simulink model "turbo_controller"  (R2025a)
settings: Solver=FixedStepAuto  StartTime=0.0  StopTime=inf  FixedStep=0.001  RelTol=1e-3
PostLoadFcn:
  | % 自动定位同目录CubeMX文件；不需要外部初始化脚本。
  | codertarget.data.setParameterValue('turbo_controller','STM32CubeMX.ProjectFile',fullfile(fileparts(get_param('turbo_controller','FileName')),'turbo_f407.ioc'));
InitFcn:
  | % 中文说明：按原控制器字段与类型创建三组接口总线；控制参数已内嵌。
  | tc_names=["EValve_Cycle" "EValve_Open" "Eblast_Cycle" "Eblast_Open" "Motor_Cycle" "Motor_Open" "EValve_Enable" "Eblast_Enable" "Motor_Enable" "SWO_Firework" "SWO_BleedAir" "EngineState" "Flag_ECUReset_Clear" "Flag_ECUReset_Save" "Flag_Reset_Enable" "Accelerator" "Nc_dem" "Nc"]; tc_types=["uint16" "uint16" "uint16" "uint16" "uint16" "uint16" "uint8" "uint8" "uint8" "uint8" "uint8" "uint8" "uint8" "uint8" "uint8" "single" "single" "single"];
  | for tc_k=1:numel(tc_names)
  |  tc_e(tc_k)=Simulink.BusElement; tc_e(tc_k).Name=char(tc_names(tc_k)); tc_e(tc_k).DataType=char(tc_types(tc_k));
  | end
  | EngineControl_Out=Simulink.Bus; EngineControl_Out.DataScope='Exported'; EngineControl_Out.Elements=tc_e;
  | clear tc_e tc_names tc_types tc_k
  | tc_names=["savedata1" "savedata2" "savedata3" "savedata4" "savedata5" "savedata6" "savedata7" "savedata8" "savedata9" "savedata10" "savedata11" "savedata12" "savedata13" "savedata14" "savedata15" "savedata16" "savedata17" "savedata18" "savedata19" "savedata20" "savedata21" "savedata22" "savedata23" "savedata24" "savedata25"]; tc_types=["single" "single" "single" "single" "single" "single" "single" "single" "single" "single" "single" "single" "single" "single" "single" "single" "single" "single" "single" "single" "single" "single" "single" "single" "single"];
  | for tc_k=1:numel(tc_names)
  |  tc_e(tc_k)=Simulink.BusElement; tc_e(tc_k).Name=char(tc_names(tc_k)); tc_e(tc_k).DataType=char(tc_types(tc_k));
  | end
  | SaveData_Out=Simulink.Bus; SaveData_Out.DataScope='Exported'; SaveData_Out.Elements=tc_e;
  | clear tc_e tc_names tc_types tc_k
  | tc_names=["senddata1" "senddata2" "senddata3" "senddata4" "senddata5" "senddata6" "senddata7" "senddata8" "senddata9" "senddata10" "senddata11" "senddata12" "senddata13" "senddata14" "senddata15" "senddata16" "senddata17" "senddata18" "senddata19" "senddata20" "senddata21" "senddata22" "senddata23" "senddata24" "senddata25" "senddata26" "senddata27" "senddata28" "senddata29"]; tc_types=["uint8" "uint8" "uint8" "uint8" "uint8" "uint8" "uint8" "uint8" "uint8" "uint8" "uint8" "uint8" "uint8" "uint8" "uint8" "uint8" "uint8" "uint8" "uint8" "uint8" "uint8" "uint8" "uint8" "uint8" "uint8" "uint8" "uint8" "uint8" "uint8"];
  | for tc_k=1:numel(tc_names)
  |  tc_e(tc_k)=Simulink.BusElement; tc_e(tc_k).Name=char(tc_names(tc_k)); tc_e(tc_k).DataType=char(tc_types(tc_k));
  | end
  | SendData_Out=Simulink.Bus; SendData_Out.DataScope='Exported'; SendData_Out.Elements=tc_e;
  | clear tc_e tc_names tc_types tc_k
  | 
  | % 以下为接口中文说明；只设置描述，不改变数值或数据类型。
  | EngineControl_Out.Description='执行控制输出（阀、电机、点火、状态及复位请求）';
  | tc_cn=["EValve_Cycle（主油阀周期计数（每计数2毫秒））" "EValve_Open（主油阀开通计数（每计数2毫秒））" "Eblast_Cycle（副油阀周期计数（每计数2毫秒））" "Eblast_Open（副油阀开通计数（每计数2毫秒））" "Motor_Cycle（起动电机周期计数）" "Motor_Open（起动电机开通计数）" "EValve_Enable（主油阀驱动使能）" "Eblast_Enable（副油阀驱动使能）" "Motor_Enable（起动电机使能）" "SWO_Firework（点火器使能（1开））" "SWO_BleedAir（引气阀使能（1开））" "EngineState（发动机状态）" "Flag_ECUReset_Clear（清除复位恢复状态请求）" "Flag_ECUReset_Save（保存复位恢复数据请求）" "Flag_Reset_Enable（处理器软件复位请求）" "Accelerator（油门／油泵给定控制量）" "Nc_dem（控制目标转速）" "Nc（发动机反馈转速（转每分））"];
  | tc_elements=EngineControl_Out.Elements;
  | for tc_k=1:numel(tc_cn)
  |  tc_elements(tc_k).Description=char(tc_cn(tc_k));
  | end
  | EngineControl_Out.Elements=tc_elements;
  | clear tc_cn tc_elements tc_k
  | SaveData_Out.Description='25项运行记录；字段含义按当前模型数据来源解释';
  | tc_cn=["savedata1（指令回显记录）" "savedata2（入口总温记录（℃））" "savedata3（电源电压记录）" "savedata4（排气温度记录（℃））" "savedata5（标定燃油压力记录）" "savedata6（副油阀占空比记录（％））" "savedata7（主油阀占空比记录（％））" "savedata8（温度修正转速记录）" "savedata9（开关输出及反馈位域）" "savedata10（物理转速记录）" "savedata11（油泵目标给定原始值）" "savedata12（起动电机占空比记录（％））" "savedata13（发动机状态码记录）" "savedata14（故障告警位域记录）" "savedata15（模型记录帧序号）" "savedata16（处理器温度记录（℃））" "savedata17（装订转速记录（沿用旧电源字段名））" "savedata18（导航高度记录）" "savedata19（飞行空速记录）" "savedata20（主阀旧记录位（恒零保留））" "savedata21（第21项保留记录（恒零））" "savedata22（保留记录项22）" "savedata23（保留记录项23）" "savedata24（保留记录项24）" "savedata25（保留记录项25）"];
  | tc_elements=SaveData_Out.Elements;
  | for tc_k=1:numel(tc_cn)
  |  tc_elements(tc_k).Description=char(tc_cn(tc_k));
  | end
  | SaveData_Out.Elements=tc_elements;
  | clear tc_cn tc_elements tc_k
  | SendData_Out.Description='29字段回传及外设命令接口；板端上位机帧只取第3至27字段';
  | tc_cn=["senddata1（回传发送允许标志（不直接上线路））" "senddata2（回传载荷长度25字节）" "senddata3（回传指令回显字节）" "senddata4（总温编码字节（℃＋80））" "senddata5（电源电压编码字节）" "senddata6（排温编码高字节）" "senddata7（排温编码低字节）" "senddata8（燃油压力编码高字节）" "senddata9（燃油压力编码低字节）" "senddata10（副油阀占空比字节（％））" "senddata11（主油阀占空比字节（％））" "senddata12（修正转速编码高字节）" "senddata13（修正转速编码低字节）" "senddata14（驱动及反馈状态位域）" "senddata15（物理转速编码高字节）" "senddata16（物理转速编码低字节）" "senddata17（油泵目标给定高字节（串口二使用））" "senddata18（油泵目标给定低字节（串口二使用））" "senddata19（起动电机占空比命令（串口一使用））" "senddata20（发动机状态码字节）" "senddata21（故障告警位域字节）" "senddata22（帧序号占位（板端另行填写））" "senddata23（处理器温度编码（℃＋50））" "senddata24（控制目标转速编码高字节）" "senddata25（控制目标转速编码低字节）" "senddata26（占位字节（板端改填实测泵速高字节））" "senddata27（占位字节（板端改填实测泵速低字节））" "senddata28（装订转速高字节（本板未发送））" "senddata29（装订转速低字节（本板未发送））"];
  | tc_elements=SendData_Out.Elements;
  | for tc_k=1:numel(tc_cn)
  |  tc_elements(tc_k).Description=char(tc_cn(tc_k));
  | end
  | SendData_Out.Elements=tc_elements;
  | clear tc_cn tc_elements tc_k
  | 
  | 
  | % FRAM模块化事务：接口类型和上电初始状态，随模型保存，无外部初始化文件。
  | clear FM_elements
  | FM_elements(1)=Simulink.BusElement;FM_elements(1).Name='phase';FM_elements(1).DataType='uint8';FM_elements(1).Dimensions=[1 1];FM_elements(1).Description='phase（当前事务阶段）';
  | FM_elements(2)=Simulink.BusElement;FM_elements(2).Name='a';FM_elements(2).DataType='uint8';FM_elements(2).Dimensions=[64 1];FM_elements(2).Description='a（启动时缓存的首区64字节）';
  | FM_elements(3)=Simulink.BusElement;FM_elements(3).Name='active';FM_elements(3).DataType='uint16';FM_elements(3).Dimensions=[1 1];FM_elements(3).Description='active（当前有效记录区地址）';
  | FM_elements(4)=Simulink.BusElement;FM_elements(4).Name='generation';FM_elements(4).DataType='uint32';FM_elements(4).Dimensions=[1 1];FM_elements(4).Description='generation（当前有效记录代号）';
  | FM_elements(5)=Simulink.BusElement;FM_elements(5).Name='record';FM_elements(5).DataType='uint8';FM_elements(5).Dimensions=[64 1];FM_elements(5).Description='record（本次冻结的待写记录）';
  | FM_elements(6)=Simulink.BusElement;FM_elements(6).Name='addr';FM_elements(6).DataType='uint16';FM_elements(6).Dimensions=[1 1];FM_elements(6).Description='addr（本次备用写入地址）';
  | FM_elements(7)=Simulink.BusElement;FM_elements(7).Name='lastSave';FM_elements(7).DataType='single';FM_elements(7).Dimensions=[1 1];FM_elements(7).Description='lastSave（上次开始保存的秒数）';
  | FM_elements(8)=Simulink.BusElement;FM_elements(8).Name='lastState';FM_elements(8).DataType='uint8';FM_elements(8).Dimensions=[1 1];FM_elements(8).Description='lastState（上次保存时的发动机状态）';
  | FM_elements(9)=Simulink.BusElement;FM_elements(9).Name='boot';FM_elements(9).DataType='boolean';FM_elements(9).Dimensions=[1 1];FM_elements(9).Description='boot（启动记录是否允许恢复）';
  | FM_elements(10)=Simulink.BusElement;FM_elements(10).Name='consumed';FM_elements(10).DataType='boolean';FM_elements(10).Dimensions=[1 1];FM_elements(10).Description='consumed（本次启动恢复通知是否已发送）';
  | FM_elements(11)=Simulink.BusElement;FM_elements(11).Name='payload';FM_elements(11).DataType='uint8';FM_elements(11).Dimensions=[20 1];FM_elements(11).Description='payload（当前20字节恢复内容）';
  | ... (+35 lines)
model workspace (MAT data in the model file):
  CRC16_Table_Reference = [0 4129 8258 12387 16516 20645 24774 28903 33032 37161 41290 45419 ... (256 elements, 256x1)]
  PE_Kaer = [0.15402 0.15402 0.12264 0.10076 0.09481 0.07601 0.07111 0.0569 0.05198 0.04926 0.05308 0.04325 ... (13 elements, 1x13)]
  PE_Nr = [21.2982 61.4260372 67.7475458 72.7394382 76.845934 80.6988798 83.8449282 86.6491912 88.9382406 89.178606 91.1938214 93.4068058 ... (13 elements, 1x13)]
  PE_Pump_Translate = 33.5999984741
  PE_RotaSpeed_Translate = 860
  PE_Taer = [0.4939154 0.4939154 0.40780982 0.34066978 0.31622756 0.30405716 0.34300244 0.26785022 0.37393554 0.23914836 0.44563948 0.31044662 ... (13 elements, 1x13)]
  PF_ACCFULLRANGE = 3360
  PF_Flag_ECUReset = 0
  PF_Flag_rx_suc = 1
  PF_Gear_Info = [40000; 45000; 50000; 55000; 57000; 59000; 60000; 61000; 61000; 61000; 61000; 61000]
  PF_K_TiaoJie = 1
  PF_Kpu = 10
  PF_MySet_Rxdata = [0 0 0 0 0 0 0 0 0 0 0 0 ... (50 elements, 50x1)]
  PF_MyUsart1_Rxdata = [0 0 0 0 0 0 0 0 0 0 0 0 ... (50 elements, 50x1)]
  PF_MyUsart2_Rxdata = [0 0 0 0 0 0 0 0 0 0 0 0 ... (50 elements, 50x1)]
  PF_Reset_Information = [0 0 0 0 0 0 0 0 0 0 0 0 ... (20 elements, 20x1)]
  PF_Sensor_X1_T4 = [0 4095]
  PF_Sensor_X2_T4 = [0 1.66666698456]
  PF_Sensor_X3_T4 = [0 504 999 1497 2010 2529 3051 3568 4076 4571 4959]
  PF_Sensor_X_P2 = [0.5 3]
  PF_Sensor_X_Poil = [0.5 3]
  PF_Sensor_X_T1t = [-50 300]
  PF_Sensor_X_Vpower = [0 3]
  PF_Sensor_X_Vpump = [0 3]
  PF_Sensor_Y1_T4 = [0 3]
  PF_Sensor_Y2_T4 = [0 5000]
  PF_Sensor_Y3_T4 = [0 100 200 300 400 500 600 700 800 900 980]
  PF_Sensor_Y_P2 = [0 1000]
  PF_Sensor_Y_Poil = [0 1000]
  PF_Sensor_Y_T1t = [-50 300]
  PF_Sensor_Y_Vpower = [0 33]
  PF_Sensor_Y_Vpump = [0 33]
  PG_CtrlMode_CloseLoop : mpt.Parameter (value not decoded)
  PG_CtrlMode_ManualAcc : mpt.Parameter (value not decoded)
  PG_CtrlMode_Origin : mpt.Parameter (value not decoded)
  PG_CtrlMode_Start : mpt.Parameter (value not decoded)
  PG_CtrlMode_Stop : mpt.Parameter (value not decoded)
  PG_ES_Clp : mpt.Parameter (value not decoded)
  PG_ES_EngStart : mpt.Parameter (value not decoded)
  PG_ES_Manual : mpt.Parameter (value not decoded)
  PG_ES_Origin : mpt.Parameter (value not decoded)
  PG_ES_Stop : mpt.Parameter (value not decoded)
  PG_Instr_BleedAirSet : mpt.Parameter (value not decoded)
  PG_Instr_CloseLoop : mpt.Parameter (value not decoded)
  PG_Instr_ECUReSet : mpt.Parameter (value not decoded)
  PG_Instr_EValveSet : mpt.Parameter (value not decoded)
  PG_Instr_EblastSet : mpt.Parameter (value not decoded)
  PG_Instr_Erase : mpt.Parameter (value not decoded)
  PG_Instr_FireWorkSet : mpt.Parameter (value not decoded)
  PG_Instr_ManualPlus : mpt.Parameter (value not decoded)
  PG_Instr_ManualrReduce : mpt.Parameter (value not decoded)
  PG_Instr_MotorSet : mpt.Parameter (value not decoded)
  PG_Instr_OilSet : mpt.Parameter (value not decoded)
  PG_Instr_SelfCheck : mpt.Parameter (value not decoded)
  PG_Instr_Start : mpt.Parameter (value not decoded)
  PG_Instr_Stop : mpt.Parameter (value not decoded)
  PG_Instr_StopZero : Simulink.Parameter (value not decoded)
  PG_Location_Air : Simulink.Parameter (value not decoded)
  PG_Location_Gnd : Simulink.Parameter (value not decoded)
  PG_ServoCtrlMode_CloseLoop : Simulink.Parameter (value not decoded)
  PG_ServoCtrlMode_CloseLoopMax : Simulink.Parameter (value not decoded)
  PG_ServoCtrlMode_CloseLoopMin : Simulink.Parameter (value not decoded)
  PG_ServoCtrlMode_ManualAcc : Simulink.Parameter (value not decoded)
  PG_ServoCtrlMode_ManualAccMax : Simulink.Parameter (value not decoded)
  PG_ServoCtrlMode_ManualAccMin : Simulink.Parameter (value not decoded)
  PG_SpeedDot_Permit : Simulink.Parameter (value not decoded)
  PL_EngineModel_Actuator = [0 10 100]
  PL_EngineModel_EngineStar_Press_P2 = [1013 1098.4 1099.144828 1099.931034 1103.613793 1162.662069 1143.793103 1131.006897 1123.186207 1117.6 1114 1111.806897 ... (127 elements, 1x127)]
  PL_EngineModel_EngineStar_RotaSpeed = [200 2000 9584 9660 10220 10240 10260 10288 10308 10368 10380 10408 ... (127 elements, 1x127)]
  PL_EngineModel_EngineStar_Temp_Exhaust = [128 129 129.1 130 131 131.1 132 133 134 134.1 135 135.1 ... (127 elements, 1x127)]
  PL_EngineModel_EngineStar_Time = [0.05 0.1 0.15 0.2 0.25 0.3 0.35 0.4 0.45 0.5 0.55 0.6 ... (127 elements, 1x127)]
  PL_EngineModel_IdleAbove_Nr = [0 21.2982 61.4260372 67.7475458 72.7394382 76.845934 80.6988798 83.8449282 86.6491912 88.9382406 89.178606 91.1938214 ... (14 elements, 1x14)]
  PL_EngineModel_IdleAbove_P2r = [0.986923266716 1.57907722675 1.81593881076 1.99358499877 2.23044658278 2.43770046879 2.65482358747 2.84233900814 3.03972366149 3.18776215149 3.25684678016 3.3950160375 ... (14 elements, 1x14)]
  PL_EngineModel_IdleAbove_Tempr = [0.0536001429337 1.07200285867 1.63301768805 1.63659103091 1.66875111667 1.72592460247 1.77595140254 1.86171163123 1.95461854565 2.03323208862 2.03323208862 2.13685903162 ... (14 elements, 1x14)]
  PL_EngineModel_IdleAbove_Ter = [0.42434128 0.42434128 0.42434128 0.30669408 0.23570008 0.22150128 0.1997974 0.23803274 0.16115638 0.24279948 0.13600422 0.31308354 ... (14 elements, 1x14)]
  PL_EngineModel_IdleAbove_Wfr = [0 10.142 23.8337 27.8905 31.9473 36.0041 40.0609 44.1177 48.1745 52.2313 52.7384 56.7952 ... (14 elements, 1x14)]
  PL_EngineModel_Press_P2 = [400 400 400 400 400 400 400 400 400 400]
  PL_EngineModel_Rotaspeed = [0 20000 96400]
  PL_EngineModel_Temp_Exhaust = [500 500 500 500 500 500 500 500 500 500]
  PL_Kaer = [0.1 0.1 0.1 0.1 0.1 0.1]
  PL_Nr = [50 60 70 80 90 100]
  PL_Taer = [0.1 0.1 0.1 0.1 0.1 0.1]
  Sig : Simulink.Signal (value not decoded)
  Ts_ms : Simulink.Parameter (value not decoded)
  false : Simulink.Parameter (value not decoded)
  true : Simulink.Parameter (value not decoded)
symbols that are objects in the model workspace (value not decoded): PG_CtrlMode_CloseLoop, PG_CtrlMode_ManualAcc, PG_CtrlMode_Origin, PG_CtrlMode_Start, PG_CtrlMode_Stop, PG_ES_Clp, PG_ES_EngStart, PG_ES_Manual, PG_ES_Origin, PG_ES_Stop, PG_Instr_BleedAirSet, PG_Instr_CloseLoop, PG_Instr_EblastSet, PG_Instr_ECUReSet, PG_Instr_Erase, PG_Instr_EValveSet, PG_Instr_FireWorkSet, PG_Instr_ManualPlus, PG_Instr_ManualrReduce, PG_Instr_MotorSet, PG_Instr_OilSet, PG_Instr_SelfCheck, PG_Instr_Start, PG_Instr_Stop, PG_Instr_StopZero, PG_ServoCtrlMode_CloseLoop, PG_ServoCtrlMode_CloseLoopMax, PG_ServoCtrlMode_CloseLoopMin, PG_ServoCtrlMode_ManualAcc, PG_ServoCtrlMode_ManualAccMax, PG_ServoCtrlMode_ManualAccMin, Ts_ms
libraries: simulink x97, stm32blockslib x10, stm32f4xxblockslib x8
(part 19 of 26)

== system turbo_controller/BoardOutput_串口封装与阀门时序/Out04_Command（电机及油泵指令）/PumpFrame（油泵指令使用原高低给定字节）_973/CRC16（只校验两个命令字节）_961 ==
  note: 【中文学习说明：CRC16查表法】
      | 一、大白话：把逐位算出的答案预先放进表里。
      | 收到每个字节后，用旧校验值和当前字节算一个表下标，
      | 直接查出结果，再与旧值左移一个字节后的部分异或。
      | 每字节只查一次表，不再进行8次逐位循环。
      |
      | 二、本模块一次处理2个数据字节。
      | 每帧校验值从0开始；逐字节循环仍按输入顺序执行。
      | 先将当前字节放到高八位，与旧CRC异或，
      | 再交给TableStep（查表更新）算出新CRC，
      | 记住新CRC后处理下一个字节，最后输出16位结果。
      |
      | 三、和参考工程逐项对应。
      | 参考写法：index=((旧CRC>>8) XOR 当前字节) AND 255。
      | 新CRC=表[index] XOR ((旧CRC<<8) AND 65535)。
      | 本图先合并字节再取高八位，得到完全相同的index。
      | 表为参考工程crc.c中的原始256项uint16数据，
      | 保存在模型工作区CRC16_Table_Reference中，
      | 所有CRC16模块使用同一份表，无需额外源文件。
      |
      | 四、协议规则没有改变。
      | 初值0、多项式0x1021、高位先处理、不作末尾异或。
      | 校验范围由外层选取，帧头和帧尾校验字节不随意加入。
      | 输出仍由外层拆成高、低字节，高字节在前。
      | 这里只计算CRC，是否采纳数据由外层校验比较决定。
      |
      | 五、记忆与循环要分清。
      | 外层逐字节循环在一次调用内处理整段数据，
      | 并非每处理一字节就等待一个采样周期。
      | CRC记忆块传递同一帧中上一个字节的结果；
      | 每次重新计算一帧时从0开始，不串用上一帧的结果。
      | 查表能发现传输错误，不能修复数据，也不是加密。
  note: 整段字节如何逐个累积CRC16
      |
      | 这里的输入Bytes是发给外设的两个命令字节，不含前五项帧头。CRC的作用是把整段字节压缩成一个16
      | 位检查值，便于接收方发现传输内容变化。
      |
      | 每帧从初始CRC=uint16(0)开始。循环一次取一个字节，把该字节乘256移到高8位，与旧CRC异或，得到
      | Merged，再交给TableStep执行查表移位。TableStep的输出成为处理下一个字节的旧CRC。
      |
      | 公式第一步是Merged=bitxor(旧CRC,当前字节×256)。整个循环结束后输出最后一次CRC，父级拆成高、
      | 低字节用于比较或发送。For Iterator中的CRC记忆是帧内累积状态，不能理解成跨帧无限累加。
      |
      | 这里用的是CRC16_Table_Reference指定的算法表，不能随意换另一种CRC表或初始值。相同字节、顺序
      | 、表和初值必须得到相同结果，双方才能校验通过。
  Bytes（待校验字节）_931 : Inport  OutDataTypeStr=uint8
  CRC（本帧累计校验值）_933 : UnitDelay  InitialCondition=uint16(0)  SampleTime=-1  HasFrameUpgradeWarning=on
  Cast（数据类型转换）_935 : DataTypeConversion  OutDataTypeStr=uint16  RndMeth=Round
  Constant（常量）_936 : Constant  Value=256  OutDataTypeStr=uint16
  CurrentByte（当前字节）_934 : Selector  InputPortWidth=2  IndexOptions=Index vector (port)  Indices=1  OutputSizes=1
  EachByte（逐字节校验）_932 : ForIterator  ResetStates=reset  IterationLimit=2  IterationVariableDataType=uint32
  HighByte（字节移到高八位）_937 : Product  Inputs=**  SaturateOnIntegerOverflow=on  OutDataTypeStr=Inherit: Same as first input
  MergeByte（并入一个字节）_938 : simulink/Logic and Bit Operations/Bitwise Operator  logicop=XOR  UseBitMask=off  NumInputPorts=2  BitMask=bin2dec('11011001')  BitMaskRealWorld=Stored Integer
      settings: LibrarySourceBlock=|
      | hdlsllib/Logic and Bit
      | Operations/Bitwise
      | Operator
  Store_uint16（按十六位无符号数保存状态）_537427 : DataTypeConversion  Description=为反馈回路显式指定原程序的状态类型，保持原状态更新节拍。  OutDataTypeStr=uint16  RndMeth=Round
  TableStep（查表更新本字节校验） : Subsystem  Description=|
      | CRC16的一个字节怎样查表更新
      | 
      | 父级已经把当前数据字节异或进旧CRC的高8位，形成Merged。本模块把这个16位数拆成“用哪项表”和“保留哪些移位结果”两部分。
      | 
      | 先取高8位：索引=floor(Merged/256)，范围0～255。用它到CRC16_Table_Reference查表；模型Selector按零基索引取值，写成MATLAB数组下标时要用索引+1。
      | 另一条支路把Merged左移一个字节，即乘256，然后只保留低16位：移位值=bitand(uint32(Merged)×256,65535)。
      | 
      | 最后将表值与移位值按位异或：
      | 新CRC=bitxor(表值,移位值)。
      | 
      | 例如Merged=十六进制1234，高8位12用于选表项，左移并截16位后为3400，再与表项异或。宽类型uint32是为了中间计算不先溢出，并不表示输出CRC变成32位。结果回到父级，继续处理下一个数据字节。
  CRC16（本帧校验结果）_960 : Outport
  wires:
  Constant（常量）_936/1 -> HighByte（字节移到高八位）_937/2  "Constant（常量）"
  Cast（数据类型转换）_935/1 -> HighByte（字节移到高八位）_937/1  "Cast（数据类型转换）"
  CurrentByte（当前字节）_934/1 -> Cast（数据类型转换）_935/1  "CurrentByte（当前字节）"
  EachByte（逐字节校验）_932/1 -> CurrentByte（当前字节）_934/2  "EachByte（逐字节校验）"
  Bytes（待校验字节）_931/1 -> CurrentByte（当前字节）_934/1  "Bytes（待校验字节）"
  TableStep（查表更新本字节校验）/1(CRC（本字节处理后的校验值）) -> CRC16（本帧校验结果）_960/1, Store_uint16（按十六位无符号数保存状态）_537427/1  "CRC16（查表更新结果）"
  MergeByte（并入一个字节）_938/1 -> TableStep（查表更新本字节校验）/1(Merged（旧校验值与当前字节异或后的数）)  "Merged（旧CRC与当前字节合并值）"
  HighByte（字节移到高八位）_937/1 -> MergeByte（并入一个字节）_938/2  "HighByte（字节移到高八位）"
  CRC（本帧累计校验值）_933/1 -> MergeByte（并入一个字节）_938/1  "CRC（本帧累计校验值）"
  Store_uint16（按十六位无符号数保存状态）_537427/1 -> CRC（本帧累计校验值）_933/1

== system turbo_controller/BoardOutput_串口封装与阀门时序/Out05_Handoff（输出交接与软件复位）/ResetService（ST官方软件复位服务）/ExecutionMode（仿真与目标运行方式）_1550 ==
  note: 仿真与目标运行方式：
      | Simulation（普通仿真）：不执行硬件复位。
      | Target（STM32目标代码）：调用 NVIC_SystemReset（系统软件复位）官方服务。
  note: 同一复位请求怎样区分电脑仿真与目标代码
      |
      | 父级ResetService已经决定这次是否执行复位；本模块只负责选择运行方式对应的实现，而不是再判断
      | 温度、油门或指令。
      |
      | Simulation是普通仿真分支，内部有意为空，因此可以在电脑运行控制模型而不执行STM32专用复位调
      | 用。
      | Target是目标代码分支，内部官方C Caller执行NVIC_SystemReset，作用于真正的控制器。
      |
      | 两条分支是运行方式选择，不应当同时作为两个控制过程解释。进入某分支不代表FRAM已经保存成功，
      | 保存事务属于另一个模块。
  Simulation（普通仿真不复位）_1548 : Subsystem  Description=|  VariantControl=(sim)
      | 电脑仿真时有意不执行硬件复位
      | 
      | 这是ExecutionMode选中的普通仿真实现。图内为空是明确设计：STM32的NVIC_SystemReset不应在普通电脑仿真里调用。
      | 
      | 外部模型仍可以计算复位请求、观察FRAM保存与控制状态，但到本分支不会真的让计算机或控制模型重新启动。要验证真实复位后的硬件启动过程，需要目标端运行，不能把空分支仿真当成已经完成硬件复位试验。
  Target（目标代码调用官方复位）_1549 : Subsystem  Description=|  VariantControl=(codegen)
      | 目标代码怎样执行真正的软件复位
      | 
      | 本分支在STM32目标代码运行方式下使用。父级已经确认复位请求，本层官方C Caller直接调用NVIC_SystemReset，触发控制器重新启动。
      | 
      | 该服务会结束当前执行过程并从硬件启动流程重新运行，不是把EngineState改为原位的普通赋值。本层不包含FRAM保存、回读校验或串口发送完成等待；这些工作必须由外层流程安排。
      | 
      | 普通电脑仿真选择另一条空实现，不执行本分支。

== system turbo_controller/CLM/ClpControl/Aim__Parameter_Calculate/Aim_AccMaxMin_Cal1 ==
  note: 把装订转速变成平缓变化的闭环目标
      |
      | 输入一项是上位机装订需求，另一项是反馈转速。本模块先让HoldFirst锁住进入闭环时的有效转速，M
      | _Rate_Limiter从这个起点逐次逼近装订值，再把目标与40000取较大值。
      |
      | 所以Nc_dem=max(变化限制后的需求,40000)。例如需求低于40000，即使限速结果更低，送控制律的目
      | 标仍是40000。这是当前模型设置，不能把上位机原始需求直接当闭环最终目标。
      |
      | 同时给出油泵给定下限700和上限8000。它们是本工程给定量的数值边界，不是转速上下限。后面的控
      | 制律和输出仲裁分别使用这些边界。
      |
      | 输出Nc_dem送PI系数计算和误差计算；Acc_Min/Acc_Max送给定限幅和故障备用控制。这里没有直接改
      | 写实际测量转速。
  S_Dem_SpeedLoad : Inport
      settings: AttributesFormatString=S_Dem_SpeedLoad（装订目标转速）
  S_Nc_Filter : Inport  Port=2
      settings: AttributesFormatString=S_Nc_Filter（滤波后的转速）
  HoldFirst : Subsystem  Description=|
      | 进入闭环时怎样避免目标突然跳变
      | 
      | 输入S_Nc_Filter是实际反馈转速，S_Dem_SpeedLoad是装订需求。两者不一定相近，如果直接把需求送误差计算，油泵给定可能出现很大瞬时变化。
      | 
      | 本模块先由Hold在首次执行时记住反馈转速，外层选择支路在反馈大于0时采用锁存值，否则继续保持此前初值。记忆支路避免每次用变化中的反馈重新设起点。
      | 接着把这个起点和装订需求送M_Rate_Limiter：每次上升140、下降100，到达目标时钳住，不越过去。
      | 
      | 例如起点40000、需求41000，前几次目标约为40140、40280、40420，最终停在41000；不会一开始直接跳到41000。
      | 输出再由父级加上最低40000限制，之后交闭环计算。这里限制的是目标变化，不是让传感器反馈也跟着被改写。
      settings: AttributesFormatString=HoldFirst（保持首次）
  MinMax : MinMax  Function=max  Inputs=2
      settings: AttributesFormatString=MinMax（最小最大值运算）
  dth = T0-288.2 : Constant  Value=40000  OutDataTypeStr=single  SampleTime=-1
      settings: AttributesFormatString=dth = T0-288.2（固定常量40000（旧名称不参与计算））
  dth = T0-288.3 : Constant  Value=700  OutDataTypeStr=single  SampleTime=-1
      settings: AttributesFormatString=dth = T0-288.3（固定常量700（旧名称不参与计算））
  dth = T0-288.5 : Constant  Value=8000  OutDataTypeStr=single  SampleTime=-1
      settings: AttributesFormatString=dth = T0-288.5（固定常量8000（旧名称不参与计算））
  Nc_dem : Outport
      settings: AttributesFormatString=Nc_dem（控制目标转速）
  Acc_Min : Outport  Port=2
      settings: AttributesFormatString=Acc_Min（油门下限）
  Acc_Max : Outport  Port=3
      settings: AttributesFormatString=Acc_Max（油门上限）
  wires:
  MinMax/1 -> Nc_dem/1
  S_Nc_Filter/1 -> HoldFirst/1(S_Nc_Filter)
  S_Dem_SpeedLoad/1 -> HoldFirst/2(S_Dem_SpeedLoad)
  HoldFirst/1(S_Dem_SpeedLoad_Limiter) -> MinMax/1
  dth = T0-288.2/1 -> MinMax/2
  dth = T0-288.3/1 -> Acc_Min/1
  dth = T0-288.5/1 -> Acc_Max/1

== system turbo_controller/CLM/ClpControl/Aim__Parameter_Calculate/PIParameter_Cal ==
  note: Kp和Ki为什么要查两遍表
      |
      | 闭环工作点会变化，同一个固定PI系数不一定适合全部转速。这里接收实际滤波转速和当前受限目标转
      | 速，对两者分别查Kp表与Ki表，共四次查表。
      |
      | 两个Kp候选取较小值，两个Ki候选也取较小值，再乘当前统一增益1：
      | Kp=min(Kp表(反馈转速),Kp表(目标转速))；
      | Ki=min(Ki表(反馈转速),Ki表(目标转速))。
      |
      | 断点覆盖约20654～60355 r/min，表中不同区段采用不同增益，断点之间按各查表块配置插值。例如某
      | 路候选Kp为0.02、另一路0.03，最终采用0.02，不把它们相加或平均。
      |
      | Kp用于误差变化量的比例项，Ki用于当前误差项。这里仅准备参数，实际增量PI在CtrlLaw执行；也不
      | 能把Ki表值单独解释成已经乘过任意新增采样时间的连续积分系数。
  S_Nc_Filter : Inport
      settings: AttributesFormatString=S_Nc_Filter（滤波后的转速）
  S_Nc_dem : Inport  Port=2
      settings: AttributesFormatString=S_Nc_dem（控制目标转速）
  Ki Lookup Table : Lookup_n-D  NumberOfTableDimensions=1  BreakpointsForDimension1=[20654 25856 30525 36143 41286 46305 51127 56000 58302 60355]  Table=single([0.00058 0.00008 0.00167 0.00156 0.00215 0.00369 0.00575 0.00684 0.00779 0.008])  ExtrapMethod=Clip  UseLastTableValue=on  InternalRulePriority=Speed  RndMeth=Simplest
      settings: AttributesFormatString=Ki Lookup Table（积分系数查找表）
  Ki Lookup Table1 : Lookup_n-D  NumberOfTableDimensions=1  BreakpointsForDimension1=[20654 25856 30525 36143 41286 46305 51127 56000 58302 60355]  Table=single([0.00058 0.00008 0.00167 0.00156 0.00215 0.00369 0.00575 0.00684 0.00779 0.008])  ExtrapMethod=Clip  UseLastTableValue=on  InternalRulePriority=Speed  RndMeth=Simplest
      settings: AttributesFormatString=Ki Lookup Table1（积分系数查找表1）
  Ki Lookup Table2 : Lookup_n-D  Commented=on  NumberOfTableDimensions=1  BreakpointsForDimension1=[22438 30016 40122 44762 49938 54926 56810 58838 59922]  Table=[0.00053 0.00086 0.0014 0.0024 0.00394 0.00582 0.00958 0.00024 0.00725]  ExtrapMethod=Clip  UseLastTableValue=on  InternalRulePriority=Speed  RndMeth=Simplest
  Kp Lookup Table : Lookup_n-D  NumberOfTableDimensions=1  BreakpointsForDimension1=[20654 25856 30525 36143 41286 46305 51127 56000 58302 60355]  Table=single([0.0058 0.0006 0.0119 0.0097 0.012 0.0185 0.0287 0.0342 0.039 0.04])  ExtrapMethod=Clip  UseLastTableValue=on  InternalRulePriority=Speed  RndMeth=Simplest
      settings: AttributesFormatString=Kp Lookup Table（比例系数查找表）
  Kp Lookup Table1 : Lookup_n-D  NumberOfTableDimensions=1  BreakpointsForDimension1=[20654 25856 30525 36143 41286 46305 51127 56000 58302 60355]  Table=single([0.0058 0.0006 0.0119 0.0097 0.012 0.0185 0.0287 0.0342 0.039 0.04])  ExtrapMethod=Clip  UseLastTableValue=on  InternalRulePriority=Speed  RndMeth=Simplest
      settings: AttributesFormatString=Kp Lookup Table1（比例系数查找表1）
  Kp Lookup Table2 : Lookup_n-D  Commented=on  NumberOfTableDimensions=1  BreakpointsForDimension1=[22438 30016 40122 44762 49938 54926 56810 58838 59922]  Table=[0.0053 0.0072 0.01 0.015 0.0219 0.0291 0.0479 0.0012 0.0363]  ExtrapMethod=Clip  UseLastTableValue=on  InternalRulePriority=Speed  RndMeth=Simplest
  Min1 : MinMax  Inputs=2
      settings: AttributesFormatString=Min1（下限1）
  Min2 : MinMax  Inputs=2
      settings: AttributesFormatString=Min2（下限2）
  Product1 : Product  Inputs=**
      settings: AttributesFormatString=Product1（乘法1）
  Product3 : Product  Inputs=**
      settings: AttributesFormatString=Product3（乘法3）
  dth = T0-288.6 : Constant  OutDataTypeStr=single  SampleTime=-1
      settings: AttributesFormatString=dth = T0-288.6（固定常量1（旧名称不参与计算））
  Kp : Outport
      settings: AttributesFormatString=Kp（比例系数）
  Ki : Outport  Port=2
      settings: AttributesFormatString=Ki（积分系数）
  wires:
  S_Nc_Filter/1 -> Ki Lookup Table/1, Kp Lookup Table/1
  Min2/1 -> Product1/2
  S_Nc_dem/1 -> Kp Lookup Table1/1, Ki Lookup Table1/1
  Min1/1 -> Product3/1
  Product3/1 -> Kp/1
  dth = T0-288.6/1 -> Product1/1, Product3/2
  Product1/1 -> Ki/1
  Kp Lookup Table/1 -> Min1/1
  Kp Lookup Table1/1 -> Min1/2
  Ki Lookup Table/1 -> Min2/1
  Ki Lookup Table1/1 -> Min2/2

== system turbo_controller/CLM/ClpControl/Fault_Process/GeneralFilter ==
  note: 让故障备用给定不要一步跳太远
      |
      | 输入Xin是备用插值给定，上下限由父级传入；Acclerator_Last是上一周期给定，Xdot_lim当前为每次
      | 10。这里的目标是平滑切到备用控制，不是测量信号滤波。
      |
      | 先把Xin限制在给定上下限，得到目标。计算目标与旧给定的差，若差的绝对值小于20，直接保持旧值
      | ，避免微小来回调整。
      | 差值达到20及以上时，根据方向从旧值加或减Xdot_lim，也就是本工程每次移动10。
      |
      | 例如旧给定1000、目标1100，本次先给1010；旧给定1000、目标1015，差值15小于20，则继续保持1000
      | 。这个模块没有按误差大小比例变化，也不是指数低通。
      |
      | 父级只有Lock_NcFailure成立才采用这一路结果。它内部的Range负责幅值约束，本层的加减负责步长
      | ，两者不能混作一种限幅。
  Xin : Inport
      settings: AttributesFormatString=Xin（输入量）
  X_ulim : Inport  Port=2
      settings: AttributesFormatString=X_ulim（输入上限）
  X_llim : Inport  Port=3
      settings: AttributesFormatString=X_llim（输入下限）
  Xdot_lim : Inport  Port=4
      settings: AttributesFormatString=Xdot_lim（变化量限值）
  Acclerator_Last : Inport  Port=5
      settings: AttributesFormatString=Acclerator_Last（油门上一周期）
  Abs : Abs  SaturateOnIntegerOverflow=off
      settings: AttributesFormatString=Abs（绝对值）
  Constant : Constant  Value=20  OutDataTypeStr=single
      settings: AttributesFormatString=Constant（常量）
  Range : Stateflow chart  Description=|  TreatAsAtomicUnit=on
      | 本实例先把故障备份曲线给出的泵编码限制在父级的X_llim～X_ulim内，再送后续死区和每拍步长处理。它只做幅值限制；差值小于20保持、否则每拍加减10在父级完成。
      | 
      | 把一个数限制在允许范围内
      | 
      | 输入包括待处理值、允许下限和允许上限。先比较是否越过上限，越过就输出上限；未超过上限时再检查下限，小于下限就输出下限；落在范围内则原样通过。恰好等于边界的值也保留。
      | 
      | 计算式：输出 = min(max(输入，下限)，上限)。
      | 例如下限为0、上限为100时，输入120输出100，输入-5输出0，输入60输出60。这里不做平均、不计算变化速度，也不记住上一拍；它只防止当前数值越界。具体边界由父子系统连入，不能把此处的输出一律理解为百分比。
      settings: AttributesFormatString=Range（限幅或范围）
  Relational Operator : RelationalOperator  Operator=<  OutDataTypeStr=boolean  InputSameDT=off
      settings: AttributesFormatString=Relational Operator（关系比较运算）
  Relational Operator1 : RelationalOperator  Operator=<  OutDataTypeStr=boolean  InputSameDT=off
      settings: AttributesFormatString=Relational Operator1（关系比较运算1）
  Sum1 : Sum  Inputs=|+-
      settings: AttributesFormatString=Sum1（加法求和1）
  Sum2 : Sum  Inputs=|++
      settings: AttributesFormatString=Sum2（加法求和2）
  Sum3 : Sum  Inputs=|+-
      settings: AttributesFormatString=Sum3（加法求和3）
  Switch : Switch  Criteria=u2 ~= 0  SaturateOnIntegerOverflow=off  InputSameDT=off
      settings: AttributesFormatString=Switch（开关选择）
  Switch1 : Switch  Criteria=u2 ~= 0  SaturateOnIntegerOverflow=off  InputSameDT=off
      settings: AttributesFormatString=Switch（开关选择）
  S_Xout : Outport
      settings: AttributesFormatString=S_Xout（输出量）
  wires:
  Xdot_lim/1 -> Sum1/2, Sum2/2
  Xin/1 -> Range/1(In)
  X_ulim/1 -> Range/2(Max)
  X_llim/1 -> Range/3(Min)
  Range/1(Out) -> Sum3/1, Relational Operator/1
  Sum3/1 -> Abs/1
  Abs/1 -> Relational Operator1/1
  Constant/1 -> Relational Operator1/2
  Switch/1 -> S_Xout/1
  Relational Operator1/1 -> Switch/2
  Acclerator_Last/1 -> Switch/1, Sum3/2, Sum1/1, Relational Operator/2, Sum2/1
  Switch1/1 -> Switch/3
  Sum2/1 -> Switch1/3
  Sum1/1 -> Switch1/1
  Relational Operator/1 -> Switch1/2

== system turbo_controller/CLM/ControlOut_Manage/Accelerator_Manage/LogicSelection3 ==
  note: 复位恢复值是否覆盖普通油泵选择
      |
      | 输入T是恢复记录的油泵给定，F是ServoCtrlOut按当前模式选出的普通给定，条件C来自Flag_ECUReset
      | _work。
      | C非零时输出T；C为零时输出F。这里是一选一，不把两个给定相加，也不做渐变。
      |
      | 例如普通给定1200、恢复值1500，许可成立时输出1500，否则1200。是否允许恢复由FPM和上游恢复解
      | 码链路决定；当前恢复许可有固定false的上游连接，不能仅凭本模块存在就认定恢复已启用。
      |
      | 输出送本层统一油泵给定端口，然后再打包为执行总线。
  C : Inport
      settings: AttributesFormatString=C（条件输入或阶段编号）
  T : Inport  Port=2
      settings: AttributesFormatString=T（温度、时间或真分支输入）
  F : Inport  Port=3
      settings: AttributesFormatString=F（假分支输入）
  Switch : Switch  Criteria=u2 ~= 0  SaturateOnIntegerOverflow=off  InputSameDT=off
      settings: AttributesFormatString=Switch（开关选择）
  Out : Outport
      settings: AttributesFormatString=Out（输出）
  wires:
  Switch/1 -> Out/1
  C/1 -> Switch/2
  T/1 -> Switch/1
  F/1 -> Switch/3

== system turbo_controller/CLM/ControlOut_Manage/SWO_Manage/Switch Case Action Subsystem ==
  note: 取出初始模式的阀门和电机控制量
      |
      | 上层已根据发动机运行模式选中本分支。本分支不再判断是否允许起动或停车，而是把这一模式给出的
      | 11个控制字段分成两组，交给后面的输出管理。
      |
      | 第一组是主油阀、副油阀和起动电机各自的“周期计数、开通计数”，共6项；第二组是这三个执行器
      | 的使能，以及点火器、引气阀的开关，共5项。这里的增益都为1，数值原样传递。
      |
      | 周期计数不是毫秒。例如阀门周期30、开通15，只表示每30个输出节拍开15拍；到板级输出以2 ms节拍
      | 执行时才对应60 ms周期、30 ms开通。使能为0时，开通计数有值也不会实际驱动。输出分别汇入控制
      | 数值总线和使能总线。
  In1 : Inport
      settings: AttributesFormatString=In1（输入1）
  Action Port : ActionPort  ActionPortLabel=case [ 1 ]:
      settings: AttributesFormatString=Action Port（动作端口）
  Bus Creator1 : BusCreator  Inputs=6
      settings: AttributesFormatString=Bus Creator1（总线创建器1）
  Bus Creator2 : BusCreator  Inputs=5
      settings: AttributesFormatString=Bus Creator2（总线创建器2）
  Bus Selector2 : BusSelector  OutputSignals=EValve_Cycle（主油阀周期计数）,EValve_Open（主油阀开通计数）,Eblast_Cycle（副油阀周期计数）,Eblast_Open（副油阀开通计数）,Motor_Cycle（起动电机周期计数）,Motor_Open（起动电机开通计数）,EValve_Enable（主油阀使能）,Eblast_Enable（副油阀使能）,Motor_Enable（起动电机使能）,SWO_Firework（点火器使能）,SWO_BleedAir（引气阀使能）
      settings: AttributesFormatString=Bus Selector2（总线选择器2）
  Gain{1..6} (6 alike) : Gain  OutDataTypeStr=uint16
      Gain1 settings: AttributesFormatString=Gain1（乘以系数1）
      Gain2 settings: AttributesFormatString=Gain2（乘以系数1）
      Gain3 settings: AttributesFormatString=Gain3（乘以系数1）
      Gain4 settings: AttributesFormatString=Gain4（乘以系数1）
      Gain5 settings: AttributesFormatString=Gain5（乘以系数1）
      Gain6 settings: AttributesFormatString=Gain6（乘以系数1）
  Gain{7..11} (5 alike) : Gain  OutDataTypeStr=uint8
      Gain10 settings: AttributesFormatString=Gain10（乘以系数1）
      Gain11 settings: AttributesFormatString=Gain11（乘以系数1）
      Gain7 settings: AttributesFormatString=Gain7（乘以系数1）
      Gain8 settings: AttributesFormatString=Gain8（乘以系数1）
      Gain9 settings: AttributesFormatString=Gain9（乘以系数1）
  Out1 : Outport
      settings: AttributesFormatString=Out1（输出1）
  Out2 : Outport  Port=2
      settings: AttributesFormatString=Out2（输出2）
  wires:
  Bus Selector2/4 -> Gain4/1  "<Eblast_Open（副油阀开通计数）>"
  Bus Selector2/5 -> Gain5/1  "<Motor_Cycle（起动电机周期计数）>"
  Bus Selector2/6 -> Gain6/1  "<Motor_Open（起动电机开通计数）>"
  Bus Selector2/7 -> Gain7/1  "<EValve_Enable（主油阀使能）>"
  Bus Selector2/8 -> Gain8/1  "<Eblast_Enable（副油阀使能）>"
  Bus Selector2/9 -> Gain9/1  "<Motor_Enable（起动电机使能）>"
  Bus Selector2/10 -> Gain10/1  "<SWO_Firework（点火器使能）>"
  Bus Selector2/1 -> Gain1/1  "<EValve_Cycle（主油阀周期计数）>"
  Bus Selector2/3 -> Gain3/1  "<Eblast_Cycle（副油阀周期计数）>"
  Bus Selector2/2 -> Gain2/1  "<EValve_Open（主油阀开通计数）>"
  Gain1/1 -> Bus Creator1/1  "EValve_Cycle（主油阀周期计数）"
  Gain2/1 -> Bus Creator1/2  "EValve_Open（主油阀开通计数）"
  Gain3/1 -> Bus Creator1/3  "Eblast_Cycle（副油阀周期计数）"
  Gain4/1 -> Bus Creator1/4  "Eblast_Open（副油阀开通计数）"
  Gain5/1 -> Bus Creator1/5  "Motor_Cycle（起动电机周期计数）"
  Gain6/1 -> Bus Creator1/6  "Motor_Open（起动电机开通计数）"
  Gain7/1 -> Bus Creator2/1  "Evalve_Enable（主油阀使能）"
  Gain8/1 -> Bus Creator2/2  "Eblast_Enable（副油阀使能）"
  Gain9/1 -> Bus Creator2/3  "Motor_Enable（起动电机使能）"
  Gain10/1 -> Bus Creator2/4  "SWO_Firework（点火器使能）"
  In1/1 -> Bus Selector2/1
  Bus Creator1/1 -> Out1/1
  Bus Creator2/1 -> Out2/1
  Bus Selector2/11 -> Gain11/1  "<SWO_BleedAir（引气阀使能）>"
  Gain11/1 -> Bus Creator2/5  "SWO_BleedAir（引气阀使能）"

== system turbo_controller/CLM/ControlOut_Manage/SWO_Manage/Switch Case Action Subsystem1 ==
  note: 取出起动模式的阀门和电机控制量
      |
      | 上层已根据发动机运行模式选中本分支。本分支不再判断是否允许起动或停车，而是把这一模式给出的
      | 11个控制字段分成两组，交给后面的输出管理。
      |
      | 第一组是主油阀、副油阀和起动电机各自的“周期计数、开通计数”，共6项；第二组是这三个执行器
      | 的使能，以及点火器、引气阀的开关，共5项。这里的增益都为1，数值原样传递。
      |
      | 周期计数不是毫秒。例如阀门周期30、开通15，只表示每30个输出节拍开15拍；到板级输出以2 ms节拍
      | 执行时才对应60 ms周期、30 ms开通。使能为0时，开通计数有值也不会实际驱动。输出分别汇入控制
      | 数值总线和使能总线。
  In1 : Inport
      settings: AttributesFormatString=In1（输入1）
  Action Port : ActionPort  ActionPortLabel=case [ 0 ]:
      settings: AttributesFormatString=Action Port（动作端口）
  Bus Creator1 : BusCreator  Inputs=6
      settings: AttributesFormatString=Bus Creator1（总线创建器1）
  Bus Creator2 : BusCreator  Inputs=5
      settings: AttributesFormatString=Bus Creator2（总线创建器2）
  Bus Selector2 : BusSelector  OutputSignals=EValve_Cycle（主油阀周期计数）,EValve_Open（主油阀开通计数）,Eblast_Cycle（副油阀周期计数）,Eblast_Open（副油阀开通计数）,Motor_Cycle（起动电机周期计数）,Motor_Open（起动电机开通计数）,EValve_Enable（主油阀使能）,Eblast_Enable（副油阀使能）,Motor_Enable（起动电机使能）,SWO_Firework（点火器使能）,SWO_BleedAir（引气阀使能）
      settings: AttributesFormatString=Bus Selector2（总线选择器2）
  Gain{1..6} (6 alike) : Gain  OutDataTypeStr=uint16
      Gain1 settings: AttributesFormatString=Gain1（乘以系数1）
      Gain2 settings: AttributesFormatString=Gain2（乘以系数1）
      Gain3 settings: AttributesFormatString=Gain3（乘以系数1）
      Gain4 settings: AttributesFormatString=Gain4（乘以系数1）
      Gain5 settings: AttributesFormatString=Gain5（乘以系数1）
      Gain6 settings: AttributesFormatString=Gain6（乘以系数1）
  Gain{7..11} (5 alike) : Gain  OutDataTypeStr=uint8
      Gain10 settings: AttributesFormatString=Gain10（乘以系数1）
      Gain11 settings: AttributesFormatString=Gain11（乘以系数1）
      Gain7 settings: AttributesFormatString=Gain7（乘以系数1）
      Gain8 settings: AttributesFormatString=Gain8（乘以系数1）
      Gain9 settings: AttributesFormatString=Gain9（乘以系数1）
  Out1 : Outport
      settings: AttributesFormatString=Out1（输出1）
  Out2 : Outport  Port=2
      settings: AttributesFormatString=Out2（输出2）
  wires:
  Bus Selector2/4 -> Gain4/1  "<Eblast_Open（副油阀开通计数）>"
  Bus Selector2/5 -> Gain5/1  "<Motor_Cycle（起动电机周期计数）>"
  Bus Selector2/6 -> Gain6/1  "<Motor_Open（起动电机开通计数）>"
  Bus Selector2/7 -> Gain7/1  "<EValve_Enable（主油阀使能）>"
  Bus Selector2/8 -> Gain8/1  "<Eblast_Enable（副油阀使能）>"
  Bus Selector2/9 -> Gain9/1  "<Motor_Enable（起动电机使能）>"
  Bus Selector2/10 -> Gain10/1  "<SWO_Firework（点火器使能）>"
  Bus Selector2/1 -> Gain1/1  "<EValve_Cycle（主油阀周期计数）>"
  Bus Selector2/3 -> Gain3/1  "<Eblast_Cycle（副油阀周期计数）>"
  Bus Selector2/2 -> Gain2/1  "<EValve_Open（主油阀开通计数）>"
  Gain1/1 -> Bus Creator1/1  "EValve_Cycle（主油阀周期计数）"
  Gain2/1 -> Bus Creator1/2  "EValve_Open（主油阀开通计数）"
  Gain3/1 -> Bus Creator1/3  "Eblast_Cycle（副油阀周期计数）"
  Gain4/1 -> Bus Creator1/4  "Eblast_Open（副油阀开通计数）"
  Gain5/1 -> Bus Creator1/5  "Motor_Cycle（起动电机周期计数）"
  Gain6/1 -> Bus Creator1/6  "Motor_Open（起动电机开通计数）"
  Gain7/1 -> Bus Creator2/1  "Evalve_Enable（主油阀使能）"
  Gain8/1 -> Bus Creator2/2  "Eblast_Enable（副油阀使能）"
  Gain9/1 -> Bus Creator2/3  "Motor_Enable（起动电机使能）"
  Gain10/1 -> Bus Creator2/4  "SWO_Firework（点火器使能）"
  In1/1 -> Bus Selector2/1
  Bus Creator1/1 -> Out1/1
  Bus Creator2/1 -> Out2/1
  Bus Selector2/11 -> Gain11/1  "<SWO_BleedAir（引气阀使能）>"
  Gain11/1 -> Bus Creator2/5  "SWO_BleedAir（引气阀使能）"

== system turbo_controller/CLM/ControlOut_Manage/SWO_Manage/Switch Case Action Subsystem2 ==
  note: 取出闭环模式的阀门和电机控制量
      |
      | 上层已根据发动机运行模式选中本分支。本分支不再判断是否允许起动或停车，而是把这一模式给出的
      | 11个控制字段分成两组，交给后面的输出管理。
      |
      | 第一组是主油阀、副油阀和起动电机各自的“周期计数、开通计数”，共6项；第二组是这三个执行器
      | 的使能，以及点火器、引气阀的开关，共5项。这里的增益都为1，数值原样传递。
      |
      | 周期计数不是毫秒。例如阀门周期30、开通15，只表示每30个输出节拍开15拍；到板级输出以2 ms节拍
      | 执行时才对应60 ms周期、30 ms开通。使能为0时，开通计数有值也不会实际驱动。输出分别汇入控制
      | 数值总线和使能总线。
  In1 : Inport
      settings: AttributesFormatString=In1（输入1）
  Action Port : ActionPort  ActionPortLabel=case [ 4 ]:
      settings: AttributesFormatString=Action Port（动作端口）
  Bus Creator1 : BusCreator  Inputs=6
      settings: AttributesFormatString=Bus Creator1（总线创建器1）
  Bus Creator2 : BusCreator  Inputs=5
      settings: AttributesFormatString=Bus Creator2（总线创建器2）
  Bus Selector2 : BusSelector  OutputSignals=EValve_Cycle（主油阀周期计数）,EValve_Open（主油阀开通计数）,Eblast_Cycle（副油阀周期计数）,Eblast_Open（副油阀开通计数）,Motor_Cycle（起动电机周期计数）,Motor_Open（起动电机开通计数）,EValve_Enable（主油阀使能）,Eblast_Enable（副油阀使能）,Motor_Enable（起动电机使能）,SWO_Firework（点火器使能）,SWO_BleedAIr（引气阀使能）
      settings: AttributesFormatString=Bus Selector2（总线选择器2）
  Gain{1..6} (6 alike) : Gain  OutDataTypeStr=uint16
      Gain1 settings: AttributesFormatString=Gain1（乘以系数1）
      Gain2 settings: AttributesFormatString=Gain2（乘以系数1）
      Gain3 settings: AttributesFormatString=Gain3（乘以系数1）
      Gain4 settings: AttributesFormatString=Gain4（乘以系数1）
      Gain5 settings: AttributesFormatString=Gain5（乘以系数1）
      Gain6 settings: AttributesFormatString=Gain6（乘以系数1）
  Gain{7..11} (5 alike) : Gain  OutDataTypeStr=uint8
      Gain10 settings: AttributesFormatString=Gain10（乘以系数1）
      Gain11 settings: AttributesFormatString=Gain11（乘以系数1）
      Gain7 settings: AttributesFormatString=Gain7（乘以系数1）
      Gain8 settings: AttributesFormatString=Gain8（乘以系数1）
      Gain9 settings: AttributesFormatString=Gain9（乘以系数1）
  Out1 : Outport
      settings: AttributesFormatString=Out1（输出1）
  Out2 : Outport  Port=2
      settings: AttributesFormatString=Out2（输出2）
  wires:
  Bus Selector2/4 -> Gain4/1  "<Eblast_Open（副油阀开通计数）>"
  Bus Selector2/5 -> Gain5/1  "<Motor_Cycle（起动电机周期计数）>"
  Bus Selector2/6 -> Gain6/1  "<Motor_Open（起动电机开通计数）>"
  Bus Selector2/7 -> Gain7/1  "<EValve_Enable（主油阀使能）>"
  Bus Selector2/8 -> Gain8/1  "<Eblast_Enable（副油阀使能）>"
  Bus Selector2/9 -> Gain9/1  "<Motor_Enable（起动电机使能）>"
  Bus Selector2/10 -> Gain10/1  "<SWO_Firework（点火器使能）>"
  Bus Selector2/1 -> Gain1/1  "<EValve_Cycle（主油阀周期计数）>"
  Bus Selector2/3 -> Gain3/1  "<Eblast_Cycle（副油阀周期计数）>"
  Bus Selector2/2 -> Gain2/1  "<EValve_Open（主油阀开通计数）>"
  Gain1/1 -> Bus Creator1/1  "EValve_Cycle（主油阀周期计数）"
  Gain2/1 -> Bus Creator1/2  "EValve_Open（主油阀开通计数）"
  Gain3/1 -> Bus Creator1/3  "Eblast_Cycle（副油阀周期计数）"
  Gain4/1 -> Bus Creator1/4  "Eblast_Open（副油阀开通计数）"
  Gain5/1 -> Bus Creator1/5  "Motor_Cycle（起动电机周期计数）"
  Gain6/1 -> Bus Creator1/6  "Motor_Open（起动电机开通计数）"
  Gain7/1 -> Bus Creator2/1  "Evalve_Enable（主油阀使能）"
  Gain8/1 -> Bus Creator2/2  "Eblast_Enable（副油阀使能）"
  Gain9/1 -> Bus Creator2/3  "Motor_Enable（起动电机使能）"
  Gain10/1 -> Bus Creator2/4  "SWO_Firework（点火器使能）"
  In1/1 -> Bus Selector2/1
  Bus Creator1/1 -> Out1/1
  Bus Creator2/1 -> Out2/1
  Bus Selector2/11 -> Gain11/1  "<SWO_BleedAIr（引气阀使能）>"
  Gain11/1 -> Bus Creator2/5  "SWO_BleedAir（引气阀使能）"

== system turbo_controller/CLM/ControlOut_Manage/SWO_Manage/Switch Case Action Subsystem3 ==
  note: 取出手动模式的阀门和电机控制量
      |
      | 上层已根据发动机运行模式选中本分支。本分支不再判断是否允许起动或停车，而是把这一模式给出的
      | 11个控制字段分成两组，交给后面的输出管理。
      |
      | 第一组是主油阀、副油阀和起动电机各自的“周期计数、开通计数”，共6项；第二组是这三个执行器
      | 的使能，以及点火器、引气阀的开关，共5项。这里的增益都为1，数值原样传递。
      |
      | 周期计数不是毫秒。例如阀门周期30、开通15，只表示每30个输出节拍开15拍；到板级输出以2 ms节拍
      | 执行时才对应60 ms周期、30 ms开通。使能为0时，开通计数有值也不会实际驱动。输出分别汇入控制
      | 数值总线和使能总线。
  In1 : Inport
      settings: AttributesFormatString=In1（输入1）
  Action Port : ActionPort  ActionPortLabel=default:
      settings: AttributesFormatString=Action Port（动作端口）
  Bus Creator1 : BusCreator  Inputs=6
      settings: AttributesFormatString=Bus Creator1（总线创建器1）
  Bus Creator2 : BusCreator  Inputs=5
      settings: AttributesFormatString=Bus Creator2（总线创建器2）
  Bus Selector2 : BusSelector  OutputSignals=SWO_BleedAir（引气阀使能）
      settings: AttributesFormatString=Bus Selector2（总线选择器2）
  Constant1 : Constant  Value=30  OutDataTypeStr=uint16  SampleTime=-1
      settings: AttributesFormatString=Constant1（常量1）
  Constant10 : Constant  Value=0  OutDataTypeStr=uint8  SampleTime=-1
      settings: AttributesFormatString=Constant10（常量10）
  Constant2 : Constant  Value=0  OutDataTypeStr=uint16  SampleTime=-1
      settings: AttributesFormatString=Constant2（常量2）
  Constant3 : Constant  Value=30  OutDataTypeStr=uint16  SampleTime=-1
      settings: AttributesFormatString=Constant3（常量3）
  Constant4 : Constant  Value=30  OutDataTypeStr=uint16  SampleTime=-1
      settings: AttributesFormatString=Constant4（常量4）
  Constant5 : Constant  OutDataTypeStr=uint8  SampleTime=-1
      settings: AttributesFormatString=Constant5（常量5）
  Constant6 : Constant  Value=0  OutDataTypeStr=uint8  SampleTime=-1
      settings: AttributesFormatString=Constant6（常量6）
  Constant7 : Constant  Value=100  OutDataTypeStr=uint16  SampleTime=-1
      settings: AttributesFormatString=Constant7（常量7）
  Constant8 : Constant  Value=0  OutDataTypeStr=uint8  SampleTime=-1
      settings: AttributesFormatString=Constant8（常量8）
  Constant9 : Constant  Value=0  OutDataTypeStr=uint16  SampleTime=-1
      settings: AttributesFormatString=Constant9（常量9）
  Gain : Gain  OutDataTypeStr=uint8
      settings: AttributesFormatString=Gain（乘以系数1）
  Out2 : Outport
      settings: AttributesFormatString=Out2（输出2）
  Out3 : Outport  Port=2
      settings: AttributesFormatString=Out3（输出3）
  wires:
  Constant1/1 -> Bus Creator1/1  "EValve_Cycle（主油阀周期计数）"
  Constant2/1 -> Bus Creator1/4  "Eblast_Open（副油阀开通计数）"
  Constant3/1 -> Bus Creator1/3  "Eblast_Cycle（副油阀周期计数）"
  Constant4/1 -> Bus Creator1/2  "EValve_Open（主油阀开通计数）"
  Constant5/1 -> Bus Creator2/1  "EValve_Enable（主油阀使能）"
  Constant6/1 -> Bus Creator2/3  "Motor_Enable（起动电机使能）"
  Constant7/1 -> Bus Creator1/5  "Motor_Cycle（起动电机周期计数）"
  Constant8/1 -> Bus Creator2/4  "SWO_Firework（点火器使能）"
  Constant9/1 -> Bus Creator1/6  "Motor_Open（起动电机开通计数）"
  Constant10/1 -> Bus Creator2/2  "Eblast_Enable（副油阀使能）"
  Bus Creator1/1 -> Out2/1
  Bus Creator2/1 -> Out3/1
  In1/1 -> Bus Selector2/1
  Bus Selector2/1 -> Gain/1  "<SWO_BleedAir（引气阀使能）>"
  Gain/1 -> Bus Creator2/5  "SWO_BleedAir（引气阀使能）"

== system turbo_controller/CLM/ControlOut_Manage/SWO_Manage/Switch Case Action Subsystem4 ==
  note: 取出停车模式的阀门和电机控制量
      |
      | 上层已根据发动机运行模式选中本分支。本分支不再判断是否允许起动或停车，而是把这一模式给出的
      | 11个控制字段分成两组，交给后面的输出管理。
      |
      | 第一组是主油阀、副油阀和起动电机各自的“周期计数、开通计数”，共6项；第二组是这三个执行器
      | 的使能，以及点火器、引气阀的开关，共5项。这里的增益都为1，数值原样传递。
      |
      | 周期计数不是毫秒。例如阀门周期30、开通15，只表示每30个输出节拍开15拍；到板级输出以2 ms节拍
      | 执行时才对应60 ms周期、30 ms开通。使能为0时，开通计数有值也不会实际驱动。输出分别汇入控制
      | 数值总线和使能总线。
  In1 : Inport
      settings: AttributesFormatString=In1（输入1）
  Action Port : ActionPort  ActionPortLabel=case [ 3 ]:
      settings: AttributesFormatString=Action Port（动作端口）
  Bus Creator1 : BusCreator  Inputs=6
      settings: AttributesFormatString=Bus Creator1（总线创建器1）
  Bus Creator2 : BusCreator  Inputs=5
      settings: AttributesFormatString=Bus Creator2（总线创建器2）
  Bus Selector2 : BusSelector  OutputSignals=EValve_Cycle（主油阀周期计数）,EValve_Open（主油阀开通计数）,Eblast_Cycle（副油阀周期计数）,Eblast_Open（副油阀开通计数）,Motor_Cycle（起动电机周期计数）,Motor_Open（起动电机开通计数）,EValve_Enable（主油阀使能）,Eblast_Enable（副油阀使能）,Motor_Enable（起动电机使能）,SWO_Firework（点火器使能）,SWO_BleedAir（引气阀使能）
      settings: AttributesFormatString=Bus Selector2（总线选择器2）
  Gain{1..6} (6 alike) : Gain  OutDataTypeStr=uint16
      Gain1 settings: AttributesFormatString=Gain1（乘以系数1）
      Gain2 settings: AttributesFormatString=Gain2（乘以系数1）
      Gain3 settings: AttributesFormatString=Gain3（乘以系数1）
      Gain4 settings: AttributesFormatString=Gain4（乘以系数1）
      Gain5 settings: AttributesFormatString=Gain5（乘以系数1）
      Gain6 settings: AttributesFormatString=Gain6（乘以系数1）
  Gain{7..11} (5 alike) : Gain  OutDataTypeStr=uint8
      Gain10 settings: AttributesFormatString=Gain10（乘以系数1）
      Gain11 settings: AttributesFormatString=Gain11（乘以系数1）
      Gain7 settings: AttributesFormatString=Gain7（乘以系数1）
      Gain8 settings: AttributesFormatString=Gain8（乘以系数1）
      Gain9 settings: AttributesFormatString=Gain9（乘以系数1）
  Out1 : Outport
      settings: AttributesFormatString=Out1（输出1）
  Out2 : Outport  Port=2
      settings: AttributesFormatString=Out2（输出2）
  wires:
  Bus Selector2/4 -> Gain4/1  "<Eblast_Open（副油阀开通计数）>"
  Bus Selector2/5 -> Gain5/1  "<Motor_Cycle（起动电机周期计数）>"
  Bus Selector2/6 -> Gain6/1  "<Motor_Open（起动电机开通计数）>"
  Bus Selector2/7 -> Gain7/1  "<EValve_Enable（主油阀使能）>"
  Bus Selector2/8 -> Gain8/1  "<Eblast_Enable（副油阀使能）>"
  Bus Selector2/9 -> Gain9/1  "<Motor_Enable（起动电机使能）>"
  Bus Selector2/10 -> Gain10/1  "<SWO_Firework（点火器使能）>"
  Bus Selector2/1 -> Gain1/1  "<EValve_Cycle（主油阀周期计数）>"
  Bus Selector2/3 -> Gain3/1  "<Eblast_Cycle（副油阀周期计数）>"
  Bus Selector2/2 -> Gain2/1  "<EValve_Open（主油阀开通计数）>"
  Gain1/1 -> Bus Creator1/1  "EValve_Cycle（主油阀周期计数）"
  Gain2/1 -> Bus Creator1/2  "EValve_Open（主油阀开通计数）"
  Gain3/1 -> Bus Creator1/3  "Eblast_Cycle（副油阀周期计数）"
  Gain4/1 -> Bus Creator1/4  "Eblast_Open（副油阀开通计数）"
  Gain5/1 -> Bus Creator1/5  "Motor_Cycle（起动电机周期计数）"
  Gain6/1 -> Bus Creator1/6  "Motor_Open（起动电机开通计数）"
  Gain7/1 -> Bus Creator2/1  "Evalve_Enable（主油阀使能）"
  Gain8/1 -> Bus Creator2/2  "Eblast_Enable（副油阀使能）"
  Gain9/1 -> Bus Creator2/3  "Motor_Enable（起动电机使能）"
  Gain10/1 -> Bus Creator2/4  "SWO_Firework（点火器使能）"
  In1/1 -> Bus Selector2/1
  Bus Creator1/1 -> Out1/1
  Bus Creator2/1 -> Out2/1
  Bus Selector2/11 -> Gain11/1  "<SWO_BleedAir（引气阀使能）>"
  Gain11/1 -> Bus Creator2/5  "SWO_BleedAir（引气阀使能）"

== system turbo_controller/CLM/Manual/ManualAcc_Min_Control/LogicSelection1 ==
  note: 在“采用新设定”和“保持旧设定”之间选择
      |
      | C是选择条件，T是条件成立时要采用的新值，F是条件不成立时保留的值。C不为0输出T，C为0输出F。
      | 这里不是三个数参与计算，也不把T、F相加。
      |
      | 在手动油泵父系统里，它用于决定是否接受本次命令。例如新设定3500、原设定3200：条件有效输出35
      | 00，条件无效仍输出3200。本模块自身没有存储，旧值由外部反馈提供。
  C : Inport
      settings: AttributesFormatString=C（条件输入或阶段编号）
  F : Inport  Port=2
      settings: AttributesFormatString=F（假分支输入）
  T : Inport  Port=3
      settings: AttributesFormatString=T（温度、时间或真分支输入）
  Switch : Switch  Criteria=u2 ~= 0  SaturateOnIntegerOverflow=off  InputSameDT=off
      settings: AttributesFormatString=Switch（开关选择）
  Out : Outport
      settings: AttributesFormatString=Out（输出）
  wires:
  Switch/1 -> Out/1
  C/1 -> Switch/2
  T/1 -> Switch/1
  F/1 -> Switch/3

== system turbo_controller/CLM/Manual/ManualAcc_Min_Control/手动加减 ==
  note: 处理手动加、减命令，并让按键作用保持一段时间
      |
      | 本分支读取命令和上次油泵给定。有效的加命令产生“旧值+100”，减命令产生“旧值-100”；其余命
      | 令保持旧值。超速保护成立时，优先走减100路径。
      |
      | Hold_500ms把触发后的操作状态维持指定时间，父级据此选择更新或保持。它的内部时间换算使用Time
      | _ms/Ts_ms；当前Ts_ms=20 ms，因此500 ms对应25次调用。名称中的500 ms表示保持窗口，不意味着每
      | 个20 ms都能无限叠加一次命令。最终值仍受父级限幅约束。
  In1 : Inport
      settings: AttributesFormatString=In1（输入1）
  In2 : Inport  Port=2
      settings: AttributesFormatString=In2（输入2）
  In3 : Inport  Port=3
      settings: AttributesFormatString=In3（输入3）
  In4 : Inport  Port=4
      settings: AttributesFormatString=In4（输入4）
  " " : Subsystem  Description=|
      | 计算一次手动增减后的候选泵给定
      | 
      | 以上次给定为基准：加命令输出旧值+100，减命令输出旧值-100，其他命令输出旧值。若Over_SpeedProtect为真，无论当前是否为加命令，都优先输出旧值-100。
      | 
      | 例如旧值3000时，加得到3100、减得到2900，超速时也得到2900。本处只计算候选值，不负责保持窗口和最终上下限；这两项在父系统完成。100是泵给定编码的一步，不是100单位油压。
  Delay : Delay  DelayLength=1
      settings: AttributesFormatString=Delay（延迟）
  Hold_500ms : Stateflow chart  Description=|  TreatAsAtomicUnit=on  RTWFcnName=Timmer  RTWFileName=EngineControl_Timmer
      | 把一次触发延长成指定时长的操作窗口
      | 
      | In为真，或上次尚在保持期间，就推进计数；否则把计数清零并令Out为假。在计数尚未达到Time_ms/Ts_ms时，Out为真并继续保持；达到门限后清计数、结束保持。
      | 
      | 当前Ts_ms=20 ms，若Time_ms=500，门限为25次调用。输入只短暂来一次，也能在后续调用继续保持。这里输出的是窗口内外的布尔状态，不是“500 ms后才出现一次”的完成脉冲。计数还在1000处封顶，防止持续累加。
      settings: AttributesFormatString=Hold_500ms（保持500毫秒）  RTWSystemCode=Reusable function  RTWFcnNameOpts=Use subsystem name  RTWFileNameOpts=User specified
  Logical Operator : Logic  AllPortsSameDT=off  OutDataTypeStr=boolean
      settings: AttributesFormatString=Logical Operator（逻辑运算）
  Logical Operator1 : Logic  Operator=OR  AllPortsSameDT=off  OutDataTypeStr=boolean
      settings: AttributesFormatString=Logical Operator1（逻辑运算1）
  Logical Operator2 : Logic  Operator=OR  AllPortsSameDT=off  OutDataTypeStr=boolean
      settings: AttributesFormatString=Logical Operator2（逻辑运算2）
  N1r_idle1 : Constant  Value=PG_Instr_ManualrReduce  OutDataTypeStr=single  SampleTime=-1
      settings: AttributesFormatString=N1r_idle1（一级转速归一化值慢车1）
  N1r_idle2 : Constant  Value=PG_Instr_ManualPlus  OutDataTypeStr=single  SampleTime=-1
      settings: AttributesFormatString=N1r_idle2（一级转速归一化值慢车2）
  Relational Operator1 : RelationalOperator  Operator===  OutDataTypeStr=boolean  InputSameDT=off
      settings: AttributesFormatString=Relational Operator1（关系比较运算1）
  Relational Operator2 : RelationalOperator  Operator===  OutDataTypeStr=boolean  InputSameDT=off
      settings: AttributesFormatString=Relational Operator2（关系比较运算2）
  Switch : Switch  Criteria=u2 ~= 0  SaturateOnIntegerOverflow=off  InputSameDT=off
      settings: AttributesFormatString=Switch（开关选择）
  Switch1 : Switch  Criteria=u2 ~= 0  SaturateOnIntegerOverflow=off  InputSameDT=off
      settings: AttributesFormatString=Switch（开关选择）
  dth = T0-288.24 : Constant  Value=500  OutDataTypeStr=single  SampleTime=-1
      settings: AttributesFormatString=dth = T0-288.24（固定常量500（旧名称不参与计算））
  Out2 : Outport
      settings: AttributesFormatString=Out2（输出2）
  wires:
  In2/1 -> Relational Operator1/1, Relational Operator2/1, " "/1(Instr)
  N1r_idle1/1 -> Relational Operator1/2
  N1r_idle2/1 -> Relational Operator2/2
  In1/1 -> Logical Operator/2
  Switch1/1 -> Out2/1  "Manual_Accelerator（手动油泵给定）"
  dth = T0-288.24/1 -> Hold_500ms/2(Time_ms)
  Switch/1 -> Switch1/3  "Manual_Accelerator（手动油泵给定）"
  Logical Operator1/1 -> Logical Operator/1
  Relational Operator2/1 -> Logical Operator1/1
  Relational Operator1/1 -> Logical Operator1/2
  Hold_500ms/1(Out) -> Delay/1
  In4/1 -> Logical Operator2/2, " "/3(Over_SpeedProtect)
  Logical Operator/1 -> Logical Operator2/1
  " "/1(Manual_Acclerator) -> Switch/1
  Logical Operator2/1 -> Switch/2, Hold_500ms/1(In)
  In3/1 -> " "/2(Acclerator_Last), Switch1/1, Switch/3
  Delay/1 -> Switch1/2
